simulink model "ferrucci299571_assign1_RW"  (R2026a)
settings: Solver=VariableStepAuto  StopTime=30  RelTol=relTol
undefined symbols (not defined in the file or in its folder): RW
libraries: fl_lib x47, nesl_utility x23, ee_lib x3
settings Model: SimulationMode=accelerator  Creator=ferru  LastModifiedBy=ferru

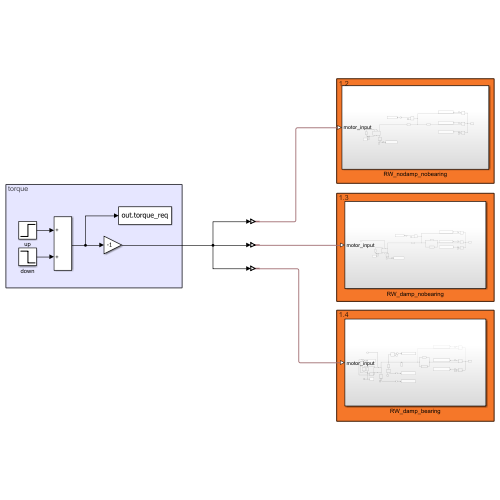
[thumbnail: Simulink's stored preview of the top-level diagram]
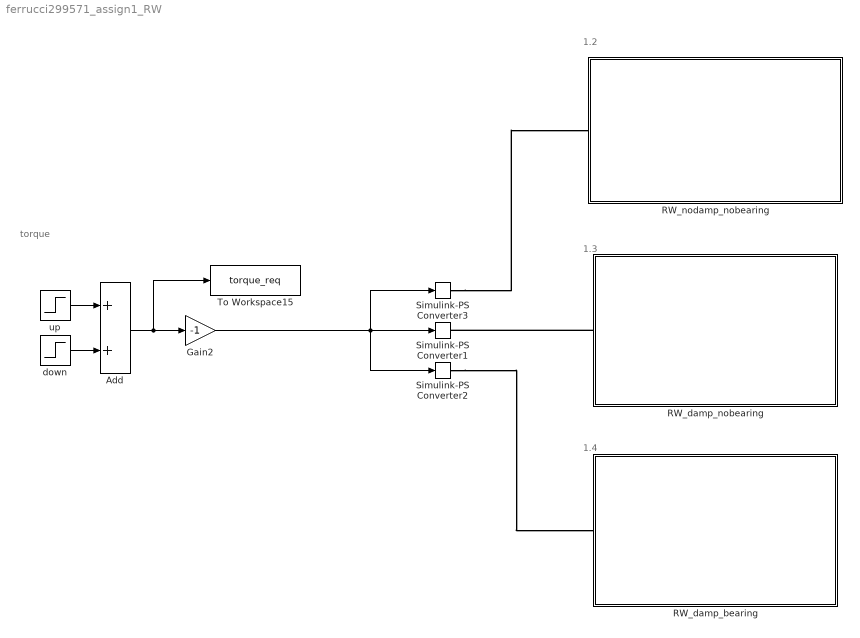
== system ferrucci299571_assign1_RW ==
  note: torque
  note: 1.2
  note: 1.3
  note: 1.4
  Add : Sum
  Gain2 : Gain  Gain=-1
  RW_damp_bearing : Subsystem
  RW_damp_nobearing : Subsystem
  RW_nodamp_nobearing : Subsystem
  Simulink-PS Converter1 : nesl_utility/Simulink-PS Converter  PhysicalDomain=network_engine_domain  SubClassName=ps_input  LeftPortType=input  RightPortType=output  PseudoPeriodic=off  Frequencies=[]  NoiseDistribution=none  NoiseParameters=[]  Unit=mN*m  AffineConversion=off  FilteringAndDerivatives=provide  SimscapeFilterOrder=1  InputFilterTimeConstant=0.001  UdotUserProvided=0
  Simulink-PS Converter2 : nesl_utility/Simulink-PS Converter  PhysicalDomain=network_engine_domain  SubClassName=ps_input  LeftPortType=input  RightPortType=output  PseudoPeriodic=off  Frequencies=[]  NoiseDistribution=none  NoiseParameters=[]  Unit=mN*m  AffineConversion=off  FilteringAndDerivatives=provide  SimscapeFilterOrder=1  InputFilterTimeConstant=0.001  UdotUserProvided=0
  Simulink-PS Converter3 : nesl_utility/Simulink-PS Converter  PhysicalDomain=network_engine_domain  SubClassName=ps_input  LeftPortType=input  RightPortType=output  PseudoPeriodic=off  Frequencies=[]  NoiseDistribution=none  NoiseParameters=[]  Unit=mN*m  AffineConversion=off  FilteringAndDerivatives=provide  SimscapeFilterOrder=1  InputFilterTimeConstant=0.001  UdotUserProvided=0
  To Workspace15 : ToWorkspace  VariableName=torque_req  SampleTime=-1
      settings: Save2DSignal=2-D array (concatenate along first dimension)
  down : Step  Time=6  FinalValue=-RW.maxTorque  SampleTime=0
  up : Step  FinalValue=RW.maxTorque  SampleTime=0
  wires:
  Gain2/1 -> Simulink-PS Converter3/1, Simulink-PS Converter2/1, Simulink-PS Converter1/1
  Add/1 -> To Workspace15/1, Gain2/1
  down/1 -> Add/2
  up/1 -> Add/1
  connections:
  Simulink-PS Converter3/RConn1 -- RW_nodamp_nobearing/LConn1
  RW_damp_nobearing/LConn1 -- Simulink-PS Converter1/RConn1
  Simulink-PS Converter2/RConn1 -- RW_damp_bearing/LConn1

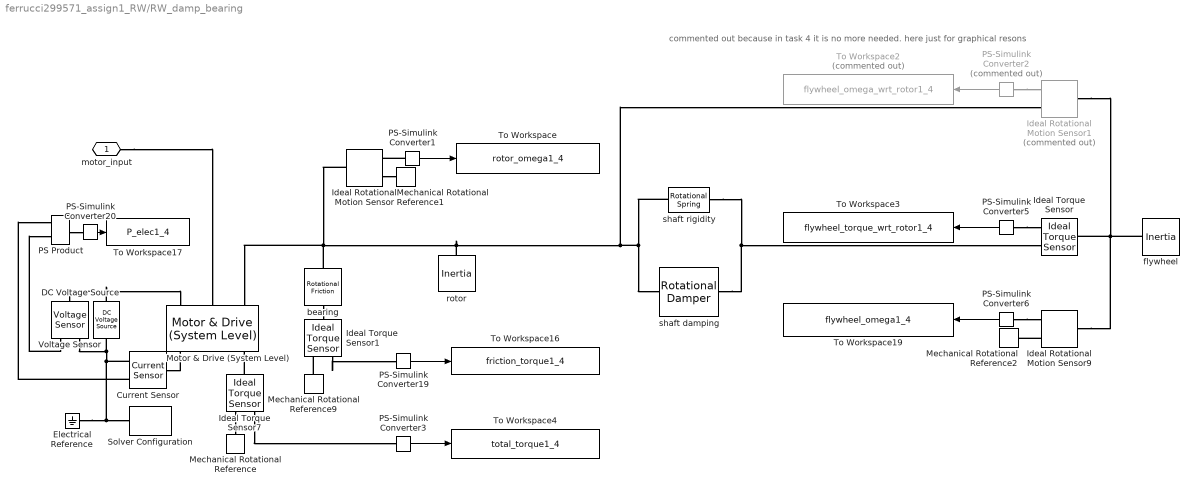
== system ferrucci299571_assign1_RW/RW_damp_bearing ==
  note: commented out because in task 4 it is no more needed. here just for graphical resons
  Current Sensor : fl_lib/Electrical/Electrical Sensors/Current Sensor
  DC Voltage Source : fl_lib/Electrical/Electrical Sources/DC Voltage Source  v0=10 V
  Electrical Reference : fl_lib/Electrical/Electrical Elements/Electrical Reference
  Ideal Rotational Motion Sensor : fl_lib/Mechanical/Mechanical Sensors/Ideal Rotational Motion Sensor  reference=foundation.enum.MeasurementReference.difference  acceleration_port=false  velocity_port=true  position_port=false  wrap_angle=false  offset=0 rad
  Ideal Rotational Motion Sensor1 : fl_lib/Mechanical/Mechanical Sensors/Ideal Rotational Motion Sensor  Commented=on  reference=foundation.enum.MeasurementReference.difference  acceleration_port=false  velocity_port=true  position_port=false  wrap_angle=false  offset=0 rad
  Ideal Rotational Motion Sensor9 : fl_lib/Mechanical/Mechanical Sensors/Ideal Rotational Motion Sensor  reference=foundation.enum.MeasurementReference.difference  acceleration_port=false  velocity_port=true  position_port=false  wrap_angle=false  offset=0 rad
  Ideal Torque Sensor : fl_lib/Mechanical/Mechanical Sensors/Ideal Torque Sensor
  Ideal Torque Sensor1 : fl_lib/Mechanical/Mechanical Sensors/Ideal Torque Sensor
  Ideal Torque Sensor7 : fl_lib/Mechanical/Mechanical Sensors/Ideal Torque Sensor
  Mechanical Rotational Reference{,1..2,9} (4 alike) : fl_lib/Mechanical/Rotational Elements/Mechanical Rotational Reference
  Motor & Drive (System Level) : ee_lib/Electromechanical/Motor & Drive (System Level)  torque_speed_param=ee.enum.electromech.envelope.tabulated  overtorque_param=ee.enum.electromech.overtorque.no  T_t=RW.torque_envelope_val mN*m  T_t_intermittent=[.36, .32, .28, 0] N*m  T_t_2D=[.09, .09, .09; .08, .08, .08; .07, .07, .07; 0, 0, 0] N*m  T_t_intermittent_2D=[.36, .36, .36; .32, .32, .32; .28, .28, .28; 0, 0, 0] N*m  w_t=RW.torque_envelope_omega rad/s  vdc_t=[6, 12, 24] V  torque_max=0.1 N*m  power_max=30 W  torque_max_intermittent=0.4 N*m  power_max_intermittent=120 W  time_overtorque=30 s  time_recover=60 s  Tc=RW.torque_control_tc s  EnableSwitch=false  losses_param=ee.enum.electromech.motorAndDrive.lossParameterization.TabulatedEfficiencyDataAsAFunctionOfSpeedAndTorque  eff=100  w_eff=3750 rpm  T_eff=0.08 N*m  Piron=0 W  Pbase=0 W  w_eff_vec=RW.efficiency_omega rad/s  T_eff_vec=RW.efficiency_torque mN*m  v_eff_vec=[100, 250, 400] V  losses_mat=[1.49, 1.67, 2.21, 3.1; .42, .69, 1.14, 2.03; .06, .24, .78, 1.68; .42, .69, 1.14, 2.03; 1.49, 1.67, 2.21, 3.1] W  efficiency_mat=RW.efficiency_mat  losses_mat_3D=ones(5, 4, 3) W  efficiency_mat_3D=95 * ones(5, 4, 3)  Res=0 Ohm  J=RW.rotor_inertia_motor kg*m^2  lam=RW.rotor_damping N*m*s/rad  speed0=0 rpm  faulted_specify=off  faulted_priority=None  faulted=0  faulted_nominal_specify=off  faulted_nominal_value=1  faulted_nominal_unit=1  isSwitchedOff_specify=off  isSwitchedOff_priority=None  isSwitchedOff=0  isSwitchedOff_nominal_specify=off  isSwitchedOff_nominal_value=1  isSwitchedOff_nominal_unit=1  torqueLimitContinuous_specify=off  torqueLimitContinuous_priority=None  torqueLimitContinuous=0 N*m  torqueLimitContinuous_nominal_specify=off  torqueLimitContinuous_nominal_value=1  torqueLimitContinuous_nominal_unit=N*m  TabulateLossesForMultipleTemperatures=false  alpha=3.93e-3 1/K  Tmeas=25 degC  TmeasVec=[25, 75, 125] degC  Tmeas2=125 degC  losses_mat_T2=[1.49, 1.74, 2.49, 3.74; .42, .67, 1.42, 2.67; .06, .31, 1.06, 2.31; .42, .67, 1.42, 2.67; 1.49, 1.74, 2.49, 3.74] W  efficiency_mat_T2=[95, 95, 95, 95; 95, 95, 95, 95; 95, 95, 95, 95; 95, 95, 95, 95; 95, 95, 95, 95]  losses_mat_3D_T2=ones(5, 4, 3) W  efficiency_mat_3D_T2=95 * ones(5, 4, 3)  lossesMatMultipleTemperatures=ones(5, 4, 3) W  efficiencyMatMultipleTemperatures=95 * ones(5, 4, 3)  lossesMat4DMultipleTemperatures=ones(5, 4, 3, 3) W  efficiencyMat4DMultipleTemperatures=95 * ones(5, 4, 3, 3)  thermal_mass=100 J/K  initial_temperature=25 degC
  PS Product : fl_lib/Physical Signals/Functions/PS Product
  PS-Simulink Converter1 : nesl_utility/PS-Simulink Converter  PhysicalDomain=network_engine_domain  SubClassName=ps_output  LeftPortType=input  RightPortType=output  PseudoPeriodic=off  Frequencies=[]  VectorFormat=inherit  Unit=rad/s  AffineConversion=off
  PS-Simulink Converter19 : nesl_utility/PS-Simulink Converter  PhysicalDomain=network_engine_domain  SubClassName=ps_output  LeftPortType=input  RightPortType=output  PseudoPeriodic=off  Frequencies=[]  VectorFormat=inherit  Unit=mN*m  AffineConversion=off
  PS-Simulink Converter2 : nesl_utility/PS-Simulink Converter  Commented=on  PhysicalDomain=network_engine_domain  SubClassName=ps_output  LeftPortType=input  RightPortType=output  PseudoPeriodic=off  Frequencies=[]  VectorFormat=inherit  Unit=rad/s  AffineConversion=off
  PS-Simulink Converter20 : nesl_utility/PS-Simulink Converter  PhysicalDomain=network_engine_domain  SubClassName=ps_output  LeftPortType=input  RightPortType=output  PseudoPeriodic=off  Frequencies=[]  VectorFormat=inherit  Unit=A*V  AffineConversion=off
  PS-Simulink Converter3 : nesl_utility/PS-Simulink Converter  PhysicalDomain=network_engine_domain  SubClassName=ps_output  LeftPortType=input  RightPortType=output  PseudoPeriodic=off  Frequencies=[]  VectorFormat=inherit  Unit=mN*m  AffineConversion=off
  PS-Simulink Converter5 : nesl_utility/PS-Simulink Converter  PhysicalDomain=network_engine_domain  SubClassName=ps_output  LeftPortType=input  RightPortType=output  PseudoPeriodic=off  Frequencies=[]  VectorFormat=inherit  Unit=mN*m  AffineConversion=off
  PS-Simulink Converter6 : nesl_utility/PS-Simulink Converter  PhysicalDomain=network_engine_domain  SubClassName=ps_output  LeftPortType=input  RightPortType=output  PseudoPeriodic=off  Frequencies=[]  VectorFormat=inherit  Unit=rad/s  AffineConversion=off
  Solver Configuration : nesl_utility/Solver Configuration  PhysicalDomain=network_engine_domain  SubClassName=solver  LeftPortType=input  RightPortType=generic  Tones=[]  Harmonics=[]  SimulateNoise=off  Profile=off  UseLocalSampling=off  EnableSwitchedLinearOptims=on  FrequencyDomain=off  UseCCode=off  RelTol=0.001  AbsTol=0.001  MinStep=1e-09  ToWorkspace=off  RevertToSquareIcSolve=off  NumHomotopyIterations=100  PhasorMode=off  PhasorModeNumHarmonics=1  ConsistencySolver=NEWTON_XTOL_AFTER_FTOL  CanonicalOrdering=CANONICAL  OptimizeIntermediates=OPTIMIZED  IndexReductionMethod=DerivativeReplacement  DoDC=off  ResidualTolerance=1e-09  ConsistencyTolSource=GLOBAL  ConsistencyAbsTol=0.001  ConsistencyRelTol=0.001  ConsistencyTolFactor=0.001  UseLocalSolver=off  LocalSolverChoice=NE_BACKWARD_EULER_ADVANCER  ResolveIndetEquations=on  FunctionEvalNumThread=1  LocalSolverSampleTime=0.001  DoFixedCost=off  MaxNonlinIter=3  MaxModeIter=2  ComputeImpulses=off  ImpulseIterations=2  LinearAlgebra=auto  LinearAlgebraNumThread=0  EquationFormulation=NE_TIME_EF  DelaysMemoryBudget=1024  AutomaticFiltering=on  FilteringTimeConstant=0.001  PartitionStorageMethod=AS_NEEDED  PartitionMemoryBudget=1024  PartitionMethod=ROBUST  MultibodyUseLocalSolver=off  MultibodyLocalSolverChoice=ODE1  MultibodyLocalSolverSampleTime=0.001
  To Workspace : ToWorkspace  VariableName=rotor_omega1_4  SampleTime=-1
      settings: Save2DSignal=2-D array (concatenate along first dimension)
  To Workspace16 : ToWorkspace  VariableName=friction_torque1_4  SampleTime=-1
      settings: Save2DSignal=2-D array (concatenate along first dimension)
  To Workspace17 : ToWorkspace  VariableName=P_elec1_4  SampleTime=-1
      settings: Save2DSignal=2-D array (concatenate along first dimension)
  To Workspace19 : ToWorkspace  VariableName=flywheel_omega1_4  SampleTime=-1
      settings: Save2DSignal=2-D array (concatenate along first dimension)
  To Workspace2 : ToWorkspace  Commented=on  VariableName=flywheel_omega_wrt_rotor1_4  SampleTime=-1
      settings: Save2DSignal=2-D array (concatenate along first dimension)
  To Workspace3 : ToWorkspace  VariableName=flywheel_torque_wrt_rotor1_4  SampleTime=-1
      settings: Save2DSignal=2-D array (concatenate along first dimension)
  To Workspace4 : ToWorkspace  VariableName=total_torque1_4  SampleTime=-1
      settings: Save2DSignal=2-D array (concatenate along first dimension)
  Voltage Sensor : fl_lib/Electrical/Electrical Sensors/Voltage Sensor
  bearing : fl_lib/Mechanical/Rotational Elements/Rotational Friction  brkwy_trq=RW.breakaway_friction_torque N*m  brkwy_vel=RW.breakaway_friction_velocity rad/s  Col_trq=RW.coulomb_friction_torque N*m  visc_coef=RW.viscous_friction_coeff N*m*s/rad  w_specify=off  w_priority=None  w=0 rad/s  w_nominal_specify=off  w_nominal_value=1  w_nominal_unit=rad/s  t_specify=off  t_priority=None  t=0 N*m  t_nominal_specify=off  t_nominal_value=1  t_nominal_unit=N*m
  flywheel : fl_lib/Mechanical/Rotational Elements/Inertia  inertia=RW.flywheel_inertia kg*m^2  num_ports=foundation.enum.numPorts2.one  w_specify=off  w_priority=High  w=0 rad/s  w_nominal_specify=off  w_nominal_value=1  w_nominal_unit=rad/s  t_specify=off  t_priority=None  t=0 N*m  t_nominal_specify=off  t_nominal_value=1  t_nominal_unit=N*m
  rotor : fl_lib/Mechanical/Rotational Elements/Inertia  inertia=RW.rotor_inertia kg*m^2  num_ports=foundation.enum.numPorts2.one  w_specify=off  w_priority=High  w=0 rad/s  w_nominal_specify=off  w_nominal_value=1  w_nominal_unit=rad/s  t_specify=off  t_priority=None  t=0 N*m  t_nominal_specify=off  t_nominal_value=1  t_nominal_unit=N*m
  shaft damping : fl_lib/Mechanical/Rotational Elements/Rotational Damper  D=RW.shaft_damping_coeff N*m*s/rad  w_specify=off  w_priority=None  w=0 rad/s  w_nominal_specify=off  w_nominal_value=1  w_nominal_unit=rad/s  t_specify=off  t_priority=None  t=0 N*m  t_nominal_specify=off  t_nominal_value=1  t_nominal_unit=N*m
  shaft rigidity : fl_lib/Mechanical/Rotational Elements/Rotational Spring  spr_rate=RW.shaft_spring_rate N*m/rad  w_specify=off  w_priority=None  w=0 rad/s  w_nominal_specify=off  w_nominal_value=1  w_nominal_unit=rad/s  t_specify=off  t_priority=None  t=0 N*m  t_nominal_specify=off  t_nominal_value=1  t_nominal_unit=N*m  phi_specify=off  phi_priority=High  phi=0 rad  phi_nominal_specify=off  phi_nominal_value=1  phi_nominal_unit=rad
  motor_input : PMIOPort  Side=Left
  wires:
  PS-Simulink Converter6/1 -> To Workspace19/1
  PS-Simulink Converter2/1 -> To Workspace2/1
  PS-Simulink Converter20/1 -> To Workspace17/1
  PS-Simulink Converter19/1 -> To Workspace16/1
  PS-Simulink Converter5/1 -> To Workspace3/1
  PS-Simulink Converter3/1 -> To Workspace4/1
  PS-Simulink Converter1/1 -> To Workspace/1
  connections:
  Ideal Torque Sensor7/RConn1 -- Mechanical Rotational Reference/LConn1
  bearing/RConn1 -- Ideal Torque Sensor1/LConn1
  Voltage Sensor/RConn1 -- PS Product/LConn2
  Ideal Torque Sensor7/RConn2 -- PS-Simulink Converter3/LConn1
  DC Voltage Source/LConn1 -- Voltage Sensor/LConn1 -- Motor & Drive (System Level)/LConn1
  bearing/LConn1 -- shaft rigidity/RConn1 -- shaft damping/RConn1 -- Ideal Rotational Motion Sensor1/RConn1 -- rotor/LConn1 -- Ideal Rotational Motion Sensor/LConn1 -- Motor & Drive (System Level)/LConn3
  Ideal Rotational Motion Sensor/RConn1 -- Mechanical Rotational Reference1/LConn1
  Ideal Torque Sensor1/RConn2 -- PS-Simulink Converter19/LConn1
  Current Sensor/RConn1 -- PS Product/LConn1
  Current Sensor/RConn2 -- Electrical Reference/LConn1 -- Solver Configuration/RConn1 -- Voltage Sensor/RConn2 -- DC Voltage Source/RConn1
  Mechanical Rotational Reference9/LConn1 -- Ideal Torque Sensor1/RConn1
  Ideal Rotational Motion Sensor9/RConn1 -- Mechanical Rotational Reference2/LConn1
  Ideal Torque Sensor/LConn1 -- Ideal Rotational Motion Sensor9/LConn1 -- flywheel/LConn1 -- Ideal Rotational Motion Sensor1/LConn1
  Ideal Torque Sensor7/LConn1 -- Motor & Drive (System Level)/RConn3
  PS-Simulink Converter1/LConn1 -- Ideal Rotational Motion Sensor/RConn2
  shaft damping/LConn1 -- shaft rigidity/LConn1 -- Ideal Torque Sensor/RConn1
  Current Sensor/LConn1 -- Motor & Drive (System Level)/RConn1
  PS-Simulink Converter2/LConn1 -- Ideal Rotational Motion Sensor1/RConn2
  motor_input/RConn1 -- Motor & Drive (System Level)/LConn2
  PS-Simulink Converter6/LConn1 -- Ideal Rotational Motion Sensor9/RConn2
  PS-Simulink Converter5/LConn1 -- Ideal Torque Sensor/RConn2
  PS Product/RConn1 -- PS-Simulink Converter20/LConn1

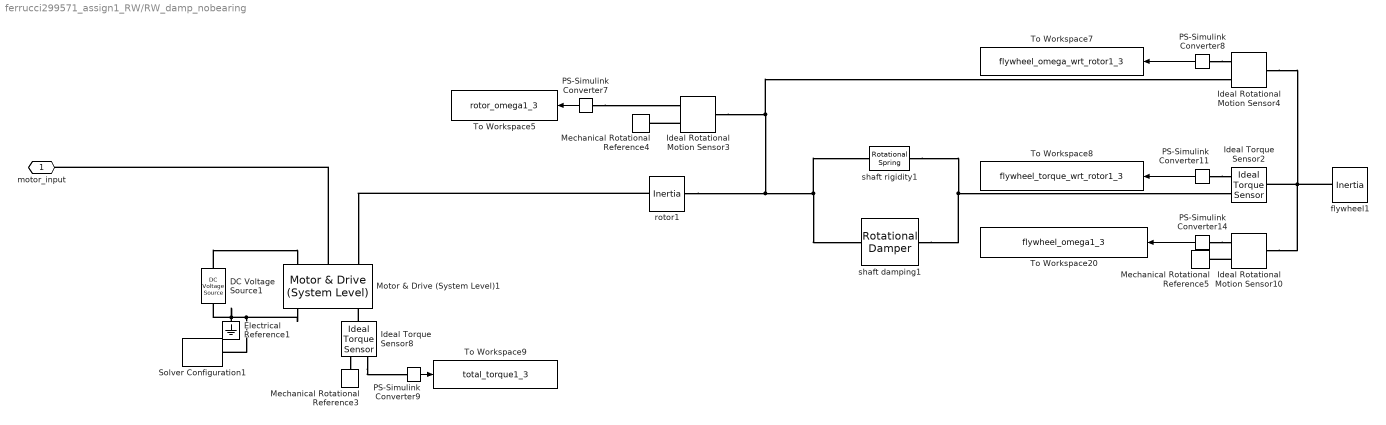
== system ferrucci299571_assign1_RW/RW_damp_nobearing ==
  DC Voltage Source1 : fl_lib/Electrical/Electrical Sources/DC Voltage Source  v0=10 V
  Electrical Reference1 : fl_lib/Electrical/Electrical Elements/Electrical Reference
  Ideal Rotational Motion Sensor10 : fl_lib/Mechanical/Mechanical Sensors/Ideal Rotational Motion Sensor  reference=foundation.enum.MeasurementReference.difference  acceleration_port=false  velocity_port=true  position_port=false  wrap_angle=false  offset=0 rad
  Ideal Rotational Motion Sensor3 : fl_lib/Mechanical/Mechanical Sensors/Ideal Rotational Motion Sensor  reference=foundation.enum.MeasurementReference.difference  acceleration_port=false  velocity_port=true  position_port=false  wrap_angle=false  offset=0 rad
  Ideal Rotational Motion Sensor4 : fl_lib/Mechanical/Mechanical Sensors/Ideal Rotational Motion Sensor  reference=foundation.enum.MeasurementReference.difference  acceleration_port=false  velocity_port=true  position_port=false  wrap_angle=false  offset=0 rad
  Ideal Torque Sensor2 : fl_lib/Mechanical/Mechanical Sensors/Ideal Torque Sensor
  Ideal Torque Sensor8 : fl_lib/Mechanical/Mechanical Sensors/Ideal Torque Sensor
  Mechanical Rotational Reference3 : fl_lib/Mechanical/Rotational Elements/Mechanical Rotational Reference
  Mechanical Rotational Reference4 : fl_lib/Mechanical/Rotational Elements/Mechanical Rotational Reference
  Mechanical Rotational Reference5 : fl_lib/Mechanical/Rotational Elements/Mechanical Rotational Reference
  Motor & Drive (System Level)1 : ee_lib/Electromechanical/Motor & Drive (System Level)  torque_speed_param=ee.enum.electromech.envelope.tabulated  overtorque_param=ee.enum.electromech.overtorque.no  T_t=RW.torque_envelope_val mN*m  T_t_intermittent=[.36, .32, .28, 0] N*m  T_t_2D=[.09, .09, .09; .08, .08, .08; .07, .07, .07; 0, 0, 0] N*m  T_t_intermittent_2D=[.36, .36, .36; .32, .32, .32; .28, .28, .28; 0, 0, 0] N*m  w_t=RW.torque_envelope_omega rad/s  vdc_t=[6, 12, 24] V  torque_max=0.1 N*m  power_max=30 W  torque_max_intermittent=0.4 N*m  power_max_intermittent=120 W  time_overtorque=30 s  time_recover=60 s  Tc=RW.torque_control_tc s  EnableSwitch=false  losses_param=ee.enum.electromech.motorAndDrive.lossParameterization.TabulatedEfficiencyDataAsAFunctionOfSpeedAndTorque  eff=100  w_eff=3750 rpm  T_eff=0.08 N*m  Piron=0 W  Pbase=0 W  w_eff_vec=RW.efficiency_omega rad/s  T_eff_vec=RW.efficiency_torque mN*m  v_eff_vec=[100, 250, 400] V  losses_mat=[1.49, 1.67, 2.21, 3.1; .42, .69, 1.14, 2.03; .06, .24, .78, 1.68; .42, .69, 1.14, 2.03; 1.49, 1.67, 2.21, 3.1] W  efficiency_mat=RW.efficiency_mat  losses_mat_3D=ones(5, 4, 3) W  efficiency_mat_3D=95 * ones(5, 4, 3)  Res=0 Ohm  J=RW.rotor_inertia_motor kg*m^2  lam=RW.rotor_damping N*m*s/rad  speed0=0 rpm  faulted_specify=off  faulted_priority=None  faulted=0  faulted_nominal_specify=off  faulted_nominal_value=1  faulted_nominal_unit=1  isSwitchedOff_specify=off  isSwitchedOff_priority=None  isSwitchedOff=0  isSwitchedOff_nominal_specify=off  isSwitchedOff_nominal_value=1  isSwitchedOff_nominal_unit=1  torqueLimitContinuous_specify=off  torqueLimitContinuous_priority=None  torqueLimitContinuous=0 N*m  torqueLimitContinuous_nominal_specify=off  torqueLimitContinuous_nominal_value=1  torqueLimitContinuous_nominal_unit=N*m  TabulateLossesForMultipleTemperatures=false  alpha=3.93e-3 1/K  Tmeas=25 degC  TmeasVec=[25, 75, 125] degC  Tmeas2=125 degC  losses_mat_T2=[1.49, 1.74, 2.49, 3.74; .42, .67, 1.42, 2.67; .06, .31, 1.06, 2.31; .42, .67, 1.42, 2.67; 1.49, 1.74, 2.49, 3.74] W  efficiency_mat_T2=[95, 95, 95, 95; 95, 95, 95, 95; 95, 95, 95, 95; 95, 95, 95, 95; 95, 95, 95, 95]  losses_mat_3D_T2=ones(5, 4, 3) W  efficiency_mat_3D_T2=95 * ones(5, 4, 3)  lossesMatMultipleTemperatures=ones(5, 4, 3) W  efficiencyMatMultipleTemperatures=95 * ones(5, 4, 3)  lossesMat4DMultipleTemperatures=ones(5, 4, 3, 3) W  efficiencyMat4DMultipleTemperatures=95 * ones(5, 4, 3, 3)  thermal_mass=100 J/K  initial_temperature=25 degC
  PS-Simulink Converter11 : nesl_utility/PS-Simulink Converter  PhysicalDomain=network_engine_domain  SubClassName=ps_output  LeftPortType=input  RightPortType=output  PseudoPeriodic=off  Frequencies=[]  VectorFormat=inherit  Unit=mN*m  AffineConversion=off
  PS-Simulink Converter14 : nesl_utility/PS-Simulink Converter  PhysicalDomain=network_engine_domain  SubClassName=ps_output  LeftPortType=input  RightPortType=output  PseudoPeriodic=off  Frequencies=[]  VectorFormat=inherit  Unit=rad/s  AffineConversion=off
  PS-Simulink Converter7 : nesl_utility/PS-Simulink Converter  PhysicalDomain=network_engine_domain  SubClassName=ps_output  LeftPortType=input  RightPortType=output  PseudoPeriodic=off  Frequencies=[]  VectorFormat=inherit  Unit=rad/s  AffineConversion=off
  PS-Simulink Converter8 : nesl_utility/PS-Simulink Converter  PhysicalDomain=network_engine_domain  SubClassName=ps_output  LeftPortType=input  RightPortType=output  PseudoPeriodic=off  Frequencies=[]  VectorFormat=inherit  Unit=rad/s  AffineConversion=off
  PS-Simulink Converter9 : nesl_utility/PS-Simulink Converter  PhysicalDomain=network_engine_domain  SubClassName=ps_output  LeftPortType=input  RightPortType=output  PseudoPeriodic=off  Frequencies=[]  VectorFormat=inherit  Unit=mN*m  AffineConversion=off
  Solver Configuration1 : nesl_utility/Solver Configuration  PhysicalDomain=network_engine_domain  SubClassName=solver  LeftPortType=input  RightPortType=generic  Tones=[]  Harmonics=[]  SimulateNoise=off  Profile=off  UseLocalSampling=off  EnableSwitchedLinearOptims=on  FrequencyDomain=off  UseCCode=off  RelTol=0.001  AbsTol=0.001  MinStep=1e-09  ToWorkspace=off  RevertToSquareIcSolve=off  NumHomotopyIterations=100  PhasorMode=off  PhasorModeNumHarmonics=1  ConsistencySolver=NEWTON_XTOL_AFTER_FTOL  CanonicalOrdering=CANONICAL  OptimizeIntermediates=OPTIMIZED  IndexReductionMethod=DerivativeReplacement  DoDC=off  ResidualTolerance=1e-09  ConsistencyTolSource=GLOBAL  ConsistencyAbsTol=0.001  ConsistencyRelTol=0.001  ConsistencyTolFactor=0.001  UseLocalSolver=off  LocalSolverChoice=NE_BACKWARD_EULER_ADVANCER  ResolveIndetEquations=on  FunctionEvalNumThread=1  LocalSolverSampleTime=0.001  DoFixedCost=off  MaxNonlinIter=3  MaxModeIter=2  ComputeImpulses=off  ImpulseIterations=2  LinearAlgebra=auto  LinearAlgebraNumThread=0  EquationFormulation=NE_TIME_EF  DelaysMemoryBudget=1024  AutomaticFiltering=on  FilteringTimeConstant=0.001  PartitionStorageMethod=AS_NEEDED  PartitionMemoryBudget=1024  PartitionMethod=ROBUST  MultibodyUseLocalSolver=off  MultibodyLocalSolverChoice=ODE1  MultibodyLocalSolverSampleTime=0.001
  To Workspace20 : ToWorkspace  VariableName=flywheel_omega1_3  SampleTime=-1
      settings: Save2DSignal=2-D array (concatenate along first dimension)
  To Workspace5 : ToWorkspace  VariableName=rotor_omega1_3  SampleTime=-1
      settings: Save2DSignal=2-D array (concatenate along first dimension)
  To Workspace7 : ToWorkspace  VariableName=flywheel_omega_wrt_rotor1_3  SampleTime=-1
      settings: Save2DSignal=2-D array (concatenate along first dimension)
  To Workspace8 : ToWorkspace  VariableName=flywheel_torque_wrt_rotor1_3  SampleTime=-1
      settings: Save2DSignal=2-D array (concatenate along first dimension)
  To Workspace9 : ToWorkspace  VariableName=total_torque1_3  SampleTime=-1
      settings: Save2DSignal=2-D array (concatenate along first dimension)
  flywheel1 : fl_lib/Mechanical/Rotational Elements/Inertia  inertia=RW.flywheel_inertia kg*m^2  num_ports=foundation.enum.numPorts2.one  w_specify=off  w_priority=High  w=0 rad/s  w_nominal_specify=off  w_nominal_value=1  w_nominal_unit=rad/s  t_specify=off  t_priority=None  t=0 N*m  t_nominal_specify=off  t_nominal_value=1  t_nominal_unit=N*m
  rotor1 : fl_lib/Mechanical/Rotational Elements/Inertia  inertia=RW.rotor_inertia kg*m^2  num_ports=foundation.enum.numPorts2.two  w_specify=off  w_priority=High  w=0 rad/s  w_nominal_specify=off  w_nominal_value=1  w_nominal_unit=rad/s  t_specify=off  t_priority=None  t=0 N*m  t_nominal_specify=off  t_nominal_value=1  t_nominal_unit=N*m
  shaft damping1 : fl_lib/Mechanical/Rotational Elements/Rotational Damper  D=RW.shaft_damping_coeff N*m*s/rad  w_specify=off  w_priority=None  w=0 rad/s  w_nominal_specify=off  w_nominal_value=1  w_nominal_unit=rad/s  t_specify=off  t_priority=None  t=0 N*m  t_nominal_specify=off  t_nominal_value=1  t_nominal_unit=N*m
  shaft rigidity1 : fl_lib/Mechanical/Rotational Elements/Rotational Spring  spr_rate=RW.shaft_spring_rate N*m/rad  w_specify=off  w_priority=None  w=0 rad/s  w_nominal_specify=off  w_nominal_value=1  w_nominal_unit=rad/s  t_specify=off  t_priority=None  t=0 N*m  t_nominal_specify=off  t_nominal_value=1  t_nominal_unit=N*m  phi_specify=off  phi_priority=High  phi=0 rad  phi_nominal_specify=off  phi_nominal_value=1  phi_nominal_unit=rad
  motor_input : PMIOPort  Side=Left
  wires:
  PS-Simulink Converter14/1 -> To Workspace20/1
  PS-Simulink Converter8/1 -> To Workspace7/1
  PS-Simulink Converter11/1 -> To Workspace8/1
  PS-Simulink Converter7/1 -> To Workspace5/1
  PS-Simulink Converter9/1 -> To Workspace9/1
  connections:
  PS-Simulink Converter11/LConn1 -- Ideal Torque Sensor2/RConn2
  Ideal Torque Sensor8/RConn2 -- PS-Simulink Converter9/LConn1
  PS-Simulink Converter7/LConn1 -- Ideal Rotational Motion Sensor3/RConn2
  Ideal Rotational Motion Sensor3/LConn1 -- Ideal Rotational Motion Sensor4/RConn1 -- shaft rigidity1/RConn1 -- shaft damping1/RConn1 -- rotor1/LConn1
  shaft rigidity1/LConn1 -- Ideal Torque Sensor2/RConn1 -- shaft damping1/LConn1
  Solver Configuration1/RConn1 -- Motor & Drive (System Level)1/RConn1 -- Electrical Reference1/LConn1 -- DC Voltage Source1/RConn1
  DC Voltage Source1/LConn1 -- Motor & Drive (System Level)1/LConn1
  flywheel1/LConn1 -- Ideal Rotational Motion Sensor10/LConn1 -- Ideal Torque Sensor2/LConn1 -- Ideal Rotational Motion Sensor4/LConn1
  Ideal Rotational Motion Sensor10/RConn1 -- Mechanical Rotational Reference5/LConn1
  Ideal Torque Sensor8/LConn1 -- Motor & Drive (System Level)1/RConn3
  Ideal Torque Sensor8/RConn1 -- Mechanical Rotational Reference3/LConn1
  PS-Simulink Converter14/LConn1 -- Ideal Rotational Motion Sensor10/RConn2
  rotor1/RConn1 -- Motor & Drive (System Level)1/LConn3
  PS-Simulink Converter8/LConn1 -- Ideal Rotational Motion Sensor4/RConn2
  Ideal Rotational Motion Sensor3/RConn1 -- Mechanical Rotational Reference4/LConn1
  Motor & Drive (System Level)1/LConn2 -- motor_input/RConn1

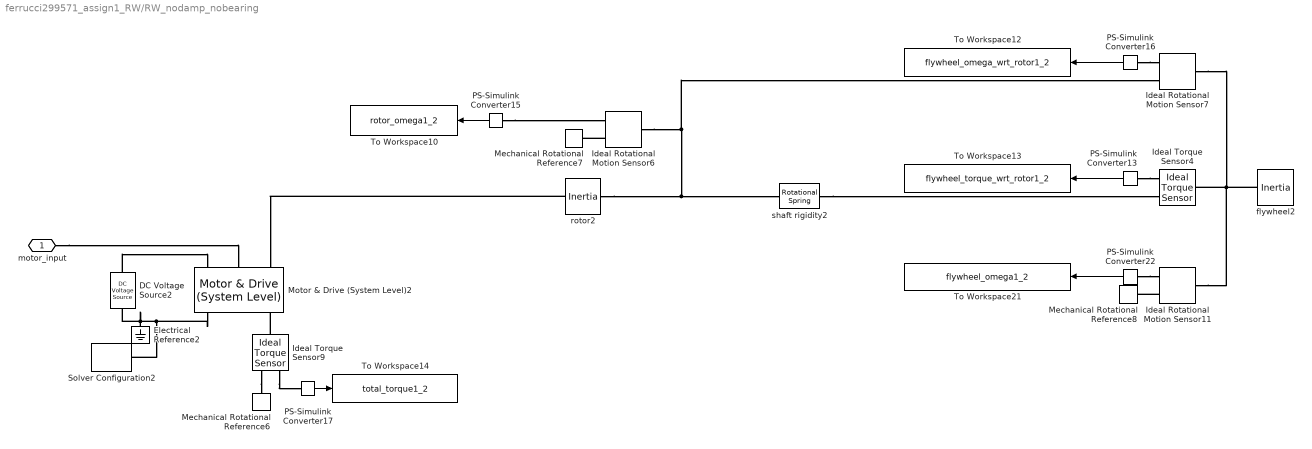
== system ferrucci299571_assign1_RW/RW_nodamp_nobearing ==
  DC Voltage Source2 : fl_lib/Electrical/Electrical Sources/DC Voltage Source  v0=10 V
  Electrical Reference2 : fl_lib/Electrical/Electrical Elements/Electrical Reference
  Ideal Rotational Motion Sensor11 : fl_lib/Mechanical/Mechanical Sensors/Ideal Rotational Motion Sensor  reference=foundation.enum.MeasurementReference.difference  acceleration_port=false  velocity_port=true  position_port=false  wrap_angle=false  offset=0 rad
  Ideal Rotational Motion Sensor6 : fl_lib/Mechanical/Mechanical Sensors/Ideal Rotational Motion Sensor  reference=foundation.enum.MeasurementReference.difference  acceleration_port=false  velocity_port=true  position_port=false  wrap_angle=false  offset=0 rad
  Ideal Rotational Motion Sensor7 : fl_lib/Mechanical/Mechanical Sensors/Ideal Rotational Motion Sensor  reference=foundation.enum.MeasurementReference.difference  acceleration_port=false  velocity_port=true  position_port=false  wrap_angle=false  offset=0 rad
  Ideal Torque Sensor4 : fl_lib/Mechanical/Mechanical Sensors/Ideal Torque Sensor
  Ideal Torque Sensor9 : fl_lib/Mechanical/Mechanical Sensors/Ideal Torque Sensor
  Mechanical Rotational Reference6 : fl_lib/Mechanical/Rotational Elements/Mechanical Rotational Reference
  Mechanical Rotational Reference7 : fl_lib/Mechanical/Rotational Elements/Mechanical Rotational Reference
  Mechanical Rotational Reference8 : fl_lib/Mechanical/Rotational Elements/Mechanical Rotational Reference
  Motor & Drive (System Level)2 : ee_lib/Electromechanical/Motor & Drive (System Level)  torque_speed_param=ee.enum.electromech.envelope.tabulated  overtorque_param=ee.enum.electromech.overtorque.no  T_t=RW.torque_envelope_val mN*m  T_t_intermittent=[.36, .32, .28, 0] N*m  T_t_2D=[.09, .09, .09; .08, .08, .08; .07, .07, .07; 0, 0, 0] N*m  T_t_intermittent_2D=[.36, .36, .36; .32, .32, .32; .28, .28, .28; 0, 0, 0] N*m  w_t=RW.torque_envelope_omega rad/s  vdc_t=[6, 12, 24] V  torque_max=0.1 N*m  power_max=30 W  torque_max_intermittent=0.4 N*m  power_max_intermittent=120 W  time_overtorque=30 s  time_recover=60 s  Tc=RW.torque_control_tc s  EnableSwitch=false  losses_param=ee.enum.electromech.motorAndDrive.lossParameterization.TabulatedEfficiencyDataAsAFunctionOfSpeedAndTorque  eff=100  w_eff=3750 rpm  T_eff=0.08 N*m  Piron=0 W  Pbase=0 W  w_eff_vec=RW.efficiency_omega rad/s  T_eff_vec=RW.efficiency_torque mN*m  v_eff_vec=[100, 250, 400] V  losses_mat=[1.49, 1.67, 2.21, 3.1; .42, .69, 1.14, 2.03; .06, .24, .78, 1.68; .42, .69, 1.14, 2.03; 1.49, 1.67, 2.21, 3.1] W  efficiency_mat=RW.efficiency_mat  losses_mat_3D=ones(5, 4, 3) W  efficiency_mat_3D=95 * ones(5, 4, 3)  Res=0 Ohm  J=RW.rotor_inertia_motor kg*m^2  lam=RW.rotor_damping N*m*s/rad  speed0=0 rpm  faulted_specify=off  faulted_priority=None  faulted=0  faulted_nominal_specify=off  faulted_nominal_value=1  faulted_nominal_unit=1  isSwitchedOff_specify=off  isSwitchedOff_priority=None  isSwitchedOff=0  isSwitchedOff_nominal_specify=off  isSwitchedOff_nominal_value=1  isSwitchedOff_nominal_unit=1  torqueLimitContinuous_specify=off  torqueLimitContinuous_priority=None  torqueLimitContinuous=0 N*m  torqueLimitContinuous_nominal_specify=off  torqueLimitContinuous_nominal_value=1  torqueLimitContinuous_nominal_unit=N*m  TabulateLossesForMultipleTemperatures=false  alpha=3.93e-3 1/K  Tmeas=25 degC  TmeasVec=[25, 75, 125] degC  Tmeas2=125 degC  losses_mat_T2=[1.49, 1.74, 2.49, 3.74; .42, .67, 1.42, 2.67; .06, .31, 1.06, 2.31; .42, .67, 1.42, 2.67; 1.49, 1.74, 2.49, 3.74] W  efficiency_mat_T2=[95, 95, 95, 95; 95, 95, 95, 95; 95, 95, 95, 95; 95, 95, 95, 95; 95, 95, 95, 95]  losses_mat_3D_T2=ones(5, 4, 3) W  efficiency_mat_3D_T2=95 * ones(5, 4, 3)  lossesMatMultipleTemperatures=ones(5, 4, 3) W  efficiencyMatMultipleTemperatures=95 * ones(5, 4, 3)  lossesMat4DMultipleTemperatures=ones(5, 4, 3, 3) W  efficiencyMat4DMultipleTemperatures=95 * ones(5, 4, 3, 3)  thermal_mass=100 J/K  initial_temperature=25 degC
  PS-Simulink Converter13 : nesl_utility/PS-Simulink Converter  PhysicalDomain=network_engine_domain  SubClassName=ps_output  LeftPortType=input  RightPortType=output  PseudoPeriodic=off  Frequencies=[]  VectorFormat=inherit  Unit=mN*m  AffineConversion=off
  PS-Simulink Converter15 : nesl_utility/PS-Simulink Converter  PhysicalDomain=network_engine_domain  SubClassName=ps_output  LeftPortType=input  RightPortType=output  PseudoPeriodic=off  Frequencies=[]  VectorFormat=inherit  Unit=rad/s  AffineConversion=off
  PS-Simulink Converter16 : nesl_utility/PS-Simulink Converter  PhysicalDomain=network_engine_domain  SubClassName=ps_output  LeftPortType=input  RightPortType=output  PseudoPeriodic=off  Frequencies=[]  VectorFormat=inherit  Unit=rad/s  AffineConversion=off
  PS-Simulink Converter17 : nesl_utility/PS-Simulink Converter  PhysicalDomain=network_engine_domain  SubClassName=ps_output  LeftPortType=input  RightPortType=output  PseudoPeriodic=off  Frequencies=[]  VectorFormat=inherit  Unit=mN*m  AffineConversion=off
  PS-Simulink Converter22 : nesl_utility/PS-Simulink Converter  PhysicalDomain=network_engine_domain  SubClassName=ps_output  LeftPortType=input  RightPortType=output  PseudoPeriodic=off  Frequencies=[]  VectorFormat=inherit  Unit=rad/s  AffineConversion=off
  Solver Configuration2 : nesl_utility/Solver Configuration  PhysicalDomain=network_engine_domain  SubClassName=solver  LeftPortType=input  RightPortType=generic  Tones=[]  Harmonics=[]  SimulateNoise=off  Profile=off  UseLocalSampling=off  EnableSwitchedLinearOptims=on  FrequencyDomain=off  UseCCode=off  RelTol=0.001  AbsTol=0.001  MinStep=1e-09  ToWorkspace=off  RevertToSquareIcSolve=off  NumHomotopyIterations=100  PhasorMode=off  PhasorModeNumHarmonics=1  ConsistencySolver=NEWTON_XTOL_AFTER_FTOL  CanonicalOrdering=CANONICAL  OptimizeIntermediates=OPTIMIZED  IndexReductionMethod=DerivativeReplacement  DoDC=off  ResidualTolerance=1e-09  ConsistencyTolSource=GLOBAL  ConsistencyAbsTol=0.001  ConsistencyRelTol=0.001  ConsistencyTolFactor=0.001  UseLocalSolver=off  LocalSolverChoice=NE_BACKWARD_EULER_ADVANCER  ResolveIndetEquations=on  FunctionEvalNumThread=1  LocalSolverSampleTime=0.001  DoFixedCost=off  MaxNonlinIter=3  MaxModeIter=2  ComputeImpulses=off  ImpulseIterations=2  LinearAlgebra=auto  LinearAlgebraNumThread=0  EquationFormulation=NE_TIME_EF  DelaysMemoryBudget=1024  AutomaticFiltering=on  FilteringTimeConstant=0.001  PartitionStorageMethod=AS_NEEDED  PartitionMemoryBudget=1024  PartitionMethod=ROBUST  MultibodyUseLocalSolver=off  MultibodyLocalSolverChoice=ODE1  MultibodyLocalSolverSampleTime=0.001
  To Workspace10 : ToWorkspace  VariableName=rotor_omega1_2  SampleTime=-1
      settings: Save2DSignal=2-D array (concatenate along first dimension)
  To Workspace12 : ToWorkspace  VariableName=flywheel_omega_wrt_rotor1_2  SampleTime=-1
      settings: Save2DSignal=2-D array (concatenate along first dimension)
  To Workspace13 : ToWorkspace  VariableName=flywheel_torque_wrt_rotor1_2  SampleTime=-1
      settings: Save2DSignal=2-D array (concatenate along first dimension)
  To Workspace14 : ToWorkspace  VariableName=total_torque1_2  SampleTime=-1
      settings: Save2DSignal=2-D array (concatenate along first dimension)
  To Workspace21 : ToWorkspace  VariableName=flywheel_omega1_2  SampleTime=-1
      settings: Save2DSignal=2-D array (concatenate along first dimension)
  flywheel2 : fl_lib/Mechanical/Rotational Elements/Inertia  inertia=RW.flywheel_inertia kg*m^2  num_ports=foundation.enum.numPorts2.one  w_specify=off  w_priority=High  w=0 rad/s  w_nominal_specify=off  w_nominal_value=1  w_nominal_unit=rad/s  t_specify=off  t_priority=None  t=0 N*m  t_nominal_specify=off  t_nominal_value=1  t_nominal_unit=N*m
  rotor2 : fl_lib/Mechanical/Rotational Elements/Inertia  inertia=RW.rotor_inertia kg*m^2  num_ports=foundation.enum.numPorts2.two  w_specify=off  w_priority=High  w=0 rad/s  w_nominal_specify=off  w_nominal_value=1  w_nominal_unit=rad/s  t_specify=off  t_priority=None  t=0 N*m  t_nominal_specify=off  t_nominal_value=1  t_nominal_unit=N*m
  shaft rigidity2 : fl_lib/Mechanical/Rotational Elements/Rotational Spring  spr_rate=RW.shaft_spring_rate N*m/rad  w_specify=off  w_priority=None  w=0 rad/s  w_nominal_specify=off  w_nominal_value=1  w_nominal_unit=rad/s  t_specify=off  t_priority=None  t=0 N*m  t_nominal_specify=off  t_nominal_value=1  t_nominal_unit=N*m  phi_specify=off  phi_priority=High  phi=0 rad  phi_nominal_specify=off  phi_nominal_value=1  phi_nominal_unit=rad
  motor_input : PMIOPort  Side=Left
  wires:
  PS-Simulink Converter15/1 -> To Workspace10/1
  PS-Simulink Converter17/1 -> To Workspace14/1
  PS-Simulink Converter22/1 -> To Workspace21/1
  PS-Simulink Converter13/1 -> To Workspace13/1
  PS-Simulink Converter16/1 -> To Workspace12/1
  connections:
  Ideal Rotational Motion Sensor6/RConn1 -- Mechanical Rotational Reference7/LConn1
  Ideal Rotational Motion Sensor11/RConn1 -- Mechanical Rotational Reference8/LConn1
  Electrical Reference2/LConn1 -- Motor & Drive (System Level)2/RConn1 -- Solver Configuration2/RConn1 -- DC Voltage Source2/RConn1
  Ideal Torque Sensor4/LConn1 -- Ideal Rotational Motion Sensor11/LConn1 -- flywheel2/LConn1 -- Ideal Rotational Motion Sensor7/LConn1
  rotor2/RConn1 -- Motor & Drive (System Level)2/LConn3
  PS-Simulink Converter16/LConn1 -- Ideal Rotational Motion Sensor7/RConn2
  PS-Simulink Converter13/LConn1 -- Ideal Torque Sensor4/RConn2
  Ideal Torque Sensor9/RConn2 -- PS-Simulink Converter17/LConn1
  DC Voltage Source2/LConn1 -- Motor & Drive (System Level)2/LConn1
  Ideal Rotational Motion Sensor6/LConn1 -- Ideal Rotational Motion Sensor7/RConn1 -- shaft rigidity2/RConn1 -- rotor2/LConn1
  Ideal Torque Sensor9/LConn1 -- Motor & Drive (System Level)2/RConn3
  Ideal Torque Sensor9/RConn1 -- Mechanical Rotational Reference6/LConn1
  shaft rigidity2/LConn1 -- Ideal Torque Sensor4/RConn1
  PS-Simulink Converter15/LConn1 -- Ideal Rotational Motion Sensor6/RConn2
  PS-Simulink Converter22/LConn1 -- Ideal Rotational Motion Sensor11/RConn2
  motor_input/RConn1 -- Motor & Drive (System Level)2/LConn2
